simulink model "Controller"  (R2023b)
settings: Solver=FixedStepDiscrete  StartTime=0.0  StopTime=10.0  FixedStep=1e-4  RelTol=1e-3
libraries: mcbcontrolslib x12, slpidlib x3, mcbpositiondecoderlib x2
settings Model: DataDictionary=Controller.sldd  Creator=84339  LastModifiedBy=84339
settings OptimizationCC: DefaultParameterBehavior=Inlined  EnhancedBackFolding=on  PassReuseOutputArgsAs=Individual arguments  ZeroExternalMemoryAtStartup=off  ZeroInternalMemoryAtStartup=off  OptimizeBlockOrder=speed  DifferentSizesBufferReuse=on  OptimizationCustomize=off  EfficientTunableParamExpr=on
settings DebuggingCC: ParameterTunabilityLossMsg=error
settings SFSimCC: MATLABDynamicMemAlloc=off
settings RTWCC: Description=Embedded Coder  SystemTargetFile=ert.tlc  EmbeddedCoderDictionary=Arch.sldd  GenCodeOnly=on  TemplateMakefile=ert_default_tmf
settings CodeAppCC: ForceParamTrailComments=on  IgnoreCustomStorageClasses=off  OperatorAnnotations=on  SimulinkDataObjDesc=on  SFDataObjDesc=on  InsertBlockDesc=on
settings ERTTargetCC: TargetLangStandard=C99 (ISO)  GenerateSampleERTMain=on  InlinedParameterPlacement=NonHierarchical  ERTCustomFileTemplate=example_file_process.tlc

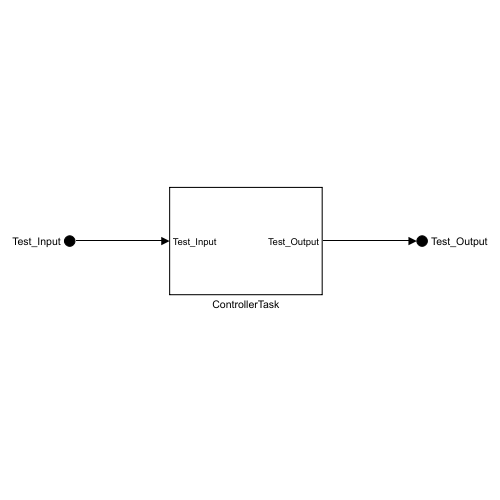
[thumbnail: Simulink's stored preview of the top-level diagram]
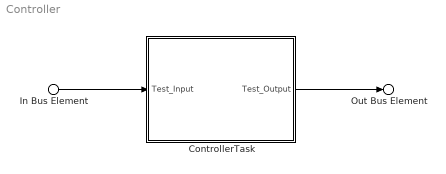
== system Controller ==
  In Bus Element : Inport  PortName=Test_Input
  ControllerTask : Subsystem
  Out Bus Element : Outport  PortName=Test_Output
  wires:
  ControllerTask/1(Test_Output) -> Out Bus Element/1
  In Bus Element/1 -> ControllerTask/1(Test_Input)

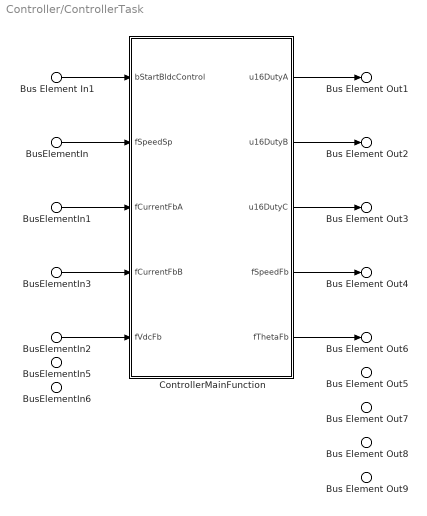
== system Controller/ControllerTask ==
  Bus Element In1 : Inport  PortName=Test_Input  Element=Input1
  BusElementIn : Inport  PortName=Test_Input  Element=Input2
  BusElementIn1 : Inport  PortName=Test_Input  Element=Input3
  BusElementIn3 : Inport  PortName=Test_Input  Element=Input4
  BusElementIn2 : Inport  PortName=Test_Input  Element=Input5
  BusElementIn5 : Inport  PortName=Test_Input  Element=Input6
  BusElementIn6 : Inport  PortName=Test_Input  Element=Input7
  ControllerMainFunction : Subsystem
  Bus Element Out1 : Outport  PortName=Test_Output  Element=Output1
  Bus Element Out2 : Outport  PortName=Test_Output  Element=Output2
  Bus Element Out3 : Outport  PortName=Test_Output  Element=Output3
  Bus Element Out4 : Outport  PortName=Test_Output  Element=Output4
  Bus Element Out5 : Outport  PortName=Test_Output  Element=Output6
  Bus Element Out7 : Outport  PortName=Test_Output  Element=Output7
  Bus Element Out8 : Outport  PortName=Test_Output  Element=Output8
  Bus Element Out9 : Outport  PortName=Test_Output  Element=Output9
  Bus Element Out6 : Outport  PortName=Test_Output  Element=Output5
  wires:
  ControllerMainFunction/1(u16DutyA) -> Bus Element Out1/1
  Bus Element In1/1 -> ControllerMainFunction/1(bStartBldcControl)
  BusElementIn/1 -> ControllerMainFunction/2(fSpeedSp)
  BusElementIn1/1 -> ControllerMainFunction/3(fCurrentFbA)
  BusElementIn3/1 -> ControllerMainFunction/4(fCurrentFbB)
  BusElementIn2/1 -> ControllerMainFunction/5(fVdcFb)
  ControllerMainFunction/2(u16DutyB) -> Bus Element Out2/1
  ControllerMainFunction/3(u16DutyC) -> Bus Element Out3/1
  ControllerMainFunction/4(fSpeedFb) -> Bus Element Out4/1
  ControllerMainFunction/5(fThetaFb) -> Bus Element Out6/1

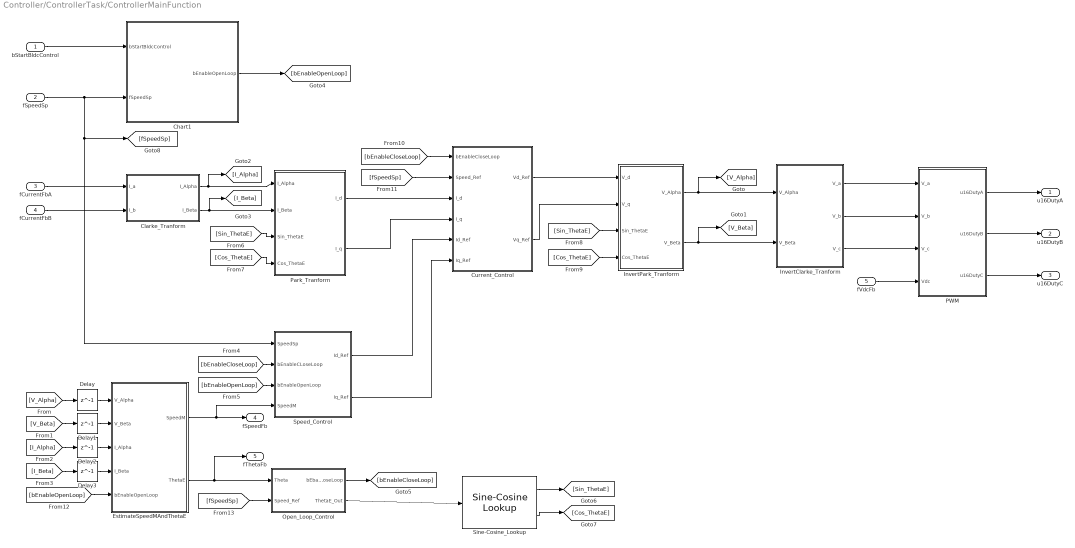
== system Controller/ControllerTask/ControllerMainFunction ==
  bStartBldcControl : Inport
  fSpeedSp : Inport  Port=2
  fCurrentFbA : Inport  Port=3
  fCurrentFbB : Inport  Port=4
  fVdcFb : Inport  Port=5
  Chart1 : Stateflow chart  TreatAsAtomicUnit=on
  Clarke_Tranform : Subsystem
  Current_Control : Subsystem
  Delay{,1..3} (4 alike) : Delay  DelayLength=1
  EstimateSpeedMAndThetaE : Subsystem
  InvertClarke_Tranform : Subsystem
  InvertPark_Tranform : Subsystem
  Open_Loop_Control : Subsystem
  PWM : Subsystem
      settings: RTWFcnNameOpts=Use subsystem name  RTWFileNameOpts=Use subsystem name
  Park_Tranform : Subsystem
  Sine-Cosine_Lookup : mcbcontrolslib/Sine-Cosine Lookup  AngleInput=Per-unit  N_points=1024
  Speed_Control : Subsystem
  u16DutyA : Outport
  u16DutyB : Outport  Port=2
  u16DutyC : Outport  Port=3
  fSpeedFb : Outport  Port=4
  fThetaFb : Outport  Port=5
  wires:
  InvertPark_Tranform/1(V_Alpha) -> [V_Alpha], InvertClarke_Tranform/1(V_Alpha)
  Delay1/1 -> EstimateSpeedMAndThetaE/2(V_Beta)
  [bEnableOpenLoop] -> Speed_Control/3(bEnableOpenLoop)
  PWM/3(u16DutyC) -> u16DutyC/1
  InvertClarke_Tranform/3(V_c) -> PWM/3(V_c)
  Delay/1 -> EstimateSpeedMAndThetaE/1(V_Alpha)
  [V_Alpha] -> Delay/1
  Speed_Control/1(Id_Ref) -> Current_Control/5(Id_Ref)
  fCurrentFbA/1 -> Clarke_Tranform/1(I_a)
  EstimateSpeedMAndThetaE/2(ThetaE) -> fThetaFb/1, Open_Loop_Control/1(Theta)
  [Cos_ThetaE] -> Park_Tranform/4(Cos_ThetaE)
  Delay2/1 -> EstimateSpeedMAndThetaE/3(I_Alpha)
  Sine-Cosine_Lookup/1 -> [Sin_ThetaE]
  Clarke_Tranform/2(I_Beta) -> Park_Tranform/2(I_Beta), [I_Beta]
  [fSpeedSp] -> Current_Control/2(Speed_Ref)
  [bEnableCloseLoop] -> Current_Control/1(bEnableCloseLoop)
  Clarke_Tranform/1(I_Alpha) -> Park_Tranform/1(I_Alpha), [I_Alpha]
  Park_Tranform/1(I_d) -> Current_Control/3(I_d)
  InvertPark_Tranform/2(V_Beta) -> [V_Beta], InvertClarke_Tranform/2(V_Beta)
  InvertClarke_Tranform/1(V_a) -> PWM/1(V_a)
  Chart1/1(bEnableOpenLoop) -> [bEnableOpenLoop]
  fCurrentFbB/1 -> Clarke_Tranform/2(I_b)
  InvertClarke_Tranform/2(V_b) -> PWM/2(V_b)
  Delay3/1 -> EstimateSpeedMAndThetaE/4(I_Beta)
  [Sin_ThetaE] -> InvertPark_Tranform/3(Sin_ThetaE)
  Park_Tranform/2(I_q) -> Current_Control/4(I_q)
  PWM/2(u16DutyB) -> u16DutyB/1
  PWM/1(u16DutyA) -> u16DutyA/1
  Open_Loop_Control/1(bEbableCloseLoop) -> [bEnableCloseLoop]
  fVdcFb/1 -> PWM/4(Vdc)
  [bEnableOpenLoop] -> EstimateSpeedMAndThetaE/5(bEnableOpenLoop)
  [V_Beta] -> Delay1/1
  [bEnableCloseLoop] -> Speed_Control/2(bEnableCLoseLoop)
  [Sin_ThetaE] -> Park_Tranform/3(Sin_ThetaE)
  [Cos_ThetaE] -> InvertPark_Tranform/4(Cos_ThetaE)
  fSpeedSp/1 -> [fSpeedSp], Speed_Control/1(SpeedSp), Chart1/2(fSpeedSp)
  EstimateSpeedMAndThetaE/1(SpeedM) -> Speed_Control/4(SpeedM), fSpeedFb/1
  Open_Loop_Control/2(ThetaE_Out) -> Sine-Cosine_Lookup/1
  Current_Control/2(Vq_Ref) -> InvertPark_Tranform/2(V_q)
  [fSpeedSp] -> Open_Loop_Control/2(Speed_Ref)
  [I_Alpha] -> Delay2/1
  [I_Beta] -> Delay3/1
  Current_Control/1(Vd_Ref) -> InvertPark_Tranform/1(V_d)
  Sine-Cosine_Lookup/2 -> [Cos_ThetaE]
  Speed_Control/2(Iq_Ref) -> Current_Control/6(Iq_Ref)
  bStartBldcControl/1 -> Chart1/1(bStartBldcControl)

== system Controller/ControllerTask/ControllerMainFunction/Clarke_Tranform ==
  I_a : Inport
  I_b : Inport  Port=2
  Clarke Transform : mcbcontrolslib/Clarke Transform  VariantControl=Variant2  PhaseInput=Two inputs  EnPowerInv=off
  I_Alpha : Outport
  I_Beta : Outport  Port=2
  wires:
  Clarke Transform/2 -> I_Beta/1
  I_a/1 -> Clarke Transform/1
  Clarke Transform/1 -> I_Alpha/1
  I_b/1 -> Clarke Transform/2

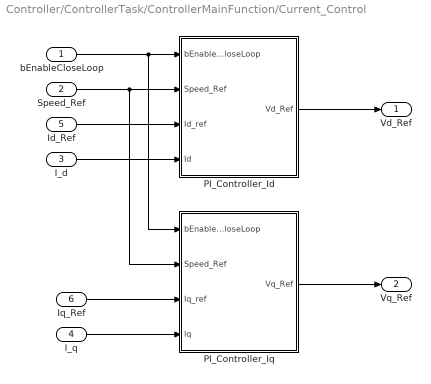
== system Controller/ControllerTask/ControllerMainFunction/Current_Control ==
  bEnableCloseLoop : Inport
  Speed_Ref : Inport  Port=2
  I_d : Inport  Port=3
  I_q : Inport  Port=4
  Id_Ref : Inport  Port=5
  Iq_Ref : Inport  Port=6
  PI_Controller_Id : Subsystem
  PI_Controller_Iq : Subsystem
  Vd_Ref : Outport
  Vq_Ref : Outport  Port=2
  wires:
  PI_Controller_Id/1(Vd_Ref) -> Vd_Ref/1
  bEnableCloseLoop/1 -> PI_Controller_Iq/1(bEnableCloseLoop), PI_Controller_Id/1(bEnableCloseLoop)
  Speed_Ref/1 -> PI_Controller_Iq/2(Speed_Ref), PI_Controller_Id/2(Speed_Ref)
  I_d/1 -> PI_Controller_Id/4(Id)
  Id_Ref/1 -> PI_Controller_Id/3(Id_ref)
  PI_Controller_Iq/1(Vq_Ref) -> Vq_Ref/1
  Iq_Ref/1 -> PI_Controller_Iq/3(Iq_ref)
  I_q/1 -> PI_Controller_Iq/4(Iq)

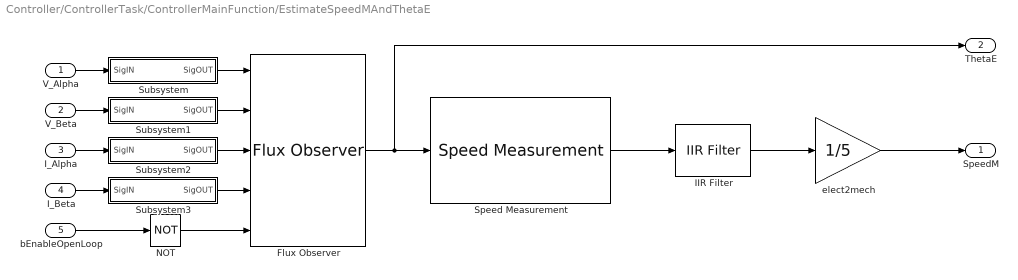
== system Controller/ControllerTask/ControllerMainFunction/EstimateSpeedMAndThetaE ==
  V_Alpha : Inport
  V_Beta : Inport  Port=2
  I_Alpha : Inport  Port=3
  I_Beta : Inport  Port=4
  bEnableOpenLoop : Inport  Port=5
  Flux Observer : mcbpositiondecoderlib/Flux Observer  MotorSelection=PMSM  DataTypeSelect=off  BlockInputUnit=Per-unit  PerUnitVoltage=24/sqrt(3)  PerUnitCurrent=7.77  PositionSelect=on  FluxSelect=off  TorqueSelect=off  PolePairs=4  StatorResistance=2.59  StatorDAxisInductance=0.5e-3  StatorLeakageInductance=0.0068  RotorLeakageInductance=0.0068  MagnetizingInductance=0.0300  CutoffFreq=3.1863  BlockSampleTime=1e-4  PositionUnit=Per-unit  PositionDatatype=single  FluxUnit=Weber  PerUnitFlux=0.1  FluxDatatype=single  TorqueUnit=Nm  PerUnitTorque=100  TorqueDatatype=single  DataType=0
  IIR Filter : mcbcontrolslib/IIR Filter  VariantControl=Low Pass Filter  VariantSelect=Low-pass  Filter_constant=0.01  advancedSettings=off  Ts=50e-6  cutOff_freq=32.1525
  NOT : Logic  Operator=NOT  IconShape=distinctive  AllPortsSameDT=off  OutDataTypeStr=boolean
  Speed Measurement : mcbpositiondecoderlib/Speed Measurement  PositionUnit=Per unit  PositionScalingDatatype=uint32  SpeedCalculationMode=Time interval for speed calculation  SampleTimeAsync=1e-4  MaximumApplicationSpeed=60000  SpeedResolution=5e-6  DelayLength=10  MaximumMeasurableSpeed=29999  MeasurableSpeedResolution=1.397e-05  SpeedUnit=Per unit based on dialog  PerUnitSpeed=2000  SpeedDataType=single
  Subsystem : Subsystem
  Subsystem1 : Subsystem
  Subsystem2 : Subsystem
  Subsystem3 : Subsystem
  elect2mech : Gain  Gain=1/5  RndMeth=Simplest  OutDataTypeStr=Inherit: Same as input
  SpeedM : Outport
  ThetaE : Outport  Port=2
  wires:
  Speed Measurement/1 -> IIR Filter/1
  Flux Observer/1 -> Speed Measurement/1, ThetaE/1
  bEnableOpenLoop/1 -> NOT/1
  NOT/1 -> Flux Observer/5
  I_Beta/1 -> Subsystem3/1(SigIN)
  I_Alpha/1 -> Subsystem2/1(SigIN)
  V_Beta/1 -> Subsystem1/1(SigIN)
  V_Alpha/1 -> Subsystem/1(SigIN)
  Subsystem/1(SigOUT) -> Flux Observer/1
  Subsystem1/1(SigOUT) -> Flux Observer/2
  Subsystem2/1(SigOUT) -> Flux Observer/3
  Subsystem3/1(SigOUT) -> Flux Observer/4
  IIR Filter/1 -> elect2mech/1
  elect2mech/1 -> SpeedM/1

== system Controller/ControllerTask/ControllerMainFunction/InvertClarke_Tranform ==
  V_Alpha : Inport
  V_Beta : Inport  Port=2
  Inverse Clarke Transform : mcbcontrolslib/Inverse Clarke Transform  PhaseInput=Two inputs  EnPowerInv=off
      settings: LibrarySourceBlock=mcblib/Controls/Math Transforms/Inverse Clarke Transform
  V_a : Outport
  V_b : Outport  Port=2
  V_c : Outport  Port=3
  wires:
  V_Alpha/1 -> Inverse Clarke Transform/1
  V_Beta/1 -> Inverse Clarke Transform/2
  Inverse Clarke Transform/2 -> V_b/1
  Inverse Clarke Transform/1 -> V_a/1
  Inverse Clarke Transform/3 -> V_c/1

== system Controller/ControllerTask/ControllerMainFunction/InvertPark_Tranform ==
  V_d : Inport
  V_q : Inport  Port=2
  Sin_ThetaE : Inport  Port=3
  Cos_ThetaE : Inport  Port=4
  Inverse Park Transform : mcbcontrolslib/Inverse Park Transform  PhaseInput=Two inputs  AxisAlignment=D-axis  ThetaInput=Sine and Cosine electrical position  AngleInput=Per-unit  N_points=1024
  V_Alpha : Outport
  V_Beta : Outport  Port=2
  wires:
  V_d/1 -> Inverse Park Transform/1
  V_q/1 -> Inverse Park Transform/2
  Sin_ThetaE/1 -> Inverse Park Transform/3
  Cos_ThetaE/1 -> Inverse Park Transform/4
  Inverse Park Transform/2 -> V_Beta/1
  Inverse Park Transform/1 -> V_Alpha/1

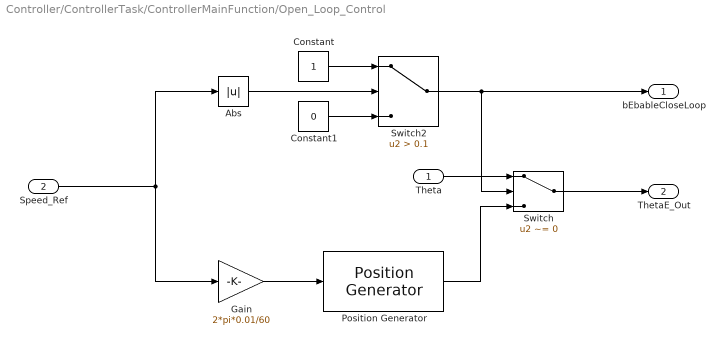
== system Controller/ControllerTask/ControllerMainFunction/Open_Loop_Control ==
  Theta : Inport
  Speed_Ref : Inport  Port=2
  Abs : Abs  SaturateOnIntegerOverflow=off
  Constant : Constant  OutDataTypeStr=boolean
  Constant1 : Constant  Value=0  OutDataTypeStr=boolean
  Gain : Gain  Gain=2*pi*0.01/60  OutDataTypeStr=Inherit: Same as input  ParamDataTypeStr=Inherit: Same as input
  Position Generator : mcbcontrolslib/Position Generator  AngleOutput=Per-unit  ExternalReset=none  Offset=0
  Switch : Switch  Criteria=u2 ~= 0  Threshold=0.1  SaturateOnIntegerOverflow=off  InputSameDT=off
  Switch2 : Switch  Criteria=u2 > Threshold  Threshold=0.1  SaturateOnIntegerOverflow=off  InputSameDT=off
  bEbableCloseLoop : Outport
  ThetaE_Out : Outport  Port=2
  wires:
  Constant1/1 -> Switch2/3
  Constant/1 -> Switch2/1
  Abs/1 -> Switch2/2
  Theta/1 -> Switch/1
  Switch/1 -> ThetaE_Out/1
  Gain/1 -> Position Generator/1
  Speed_Ref/1 -> Abs/1, Gain/1
  Switch2/1 -> Switch/2, bEbableCloseLoop/1
  Position Generator/1 -> Switch/3

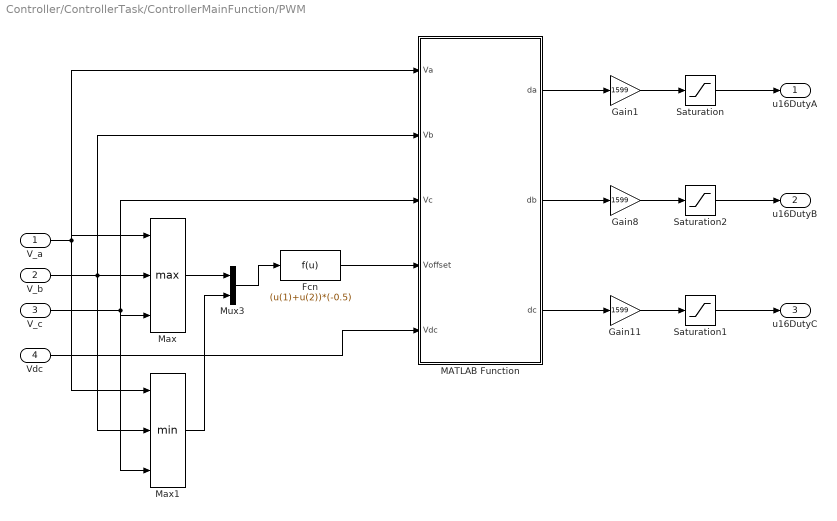
== system Controller/ControllerTask/ControllerMainFunction/PWM ==
  V_a : Inport
  V_b : Inport  Port=2
  V_c : Inport  Port=3
  Vdc : Inport  Port=4
  Fcn : Fcn  Expr=(u(1)+u(2))*(-0.5)
  Gain1 : Gain  Gain=1599  OutDataTypeStr=uint16
  Gain11 : Gain  Gain=1599  OutDataTypeStr=uint16
  Gain8 : Gain  Gain=1599  OutDataTypeStr=uint16
  MATLAB Function : MATLAB Function  TreatAsAtomicUnit=on
  Max : MinMax  Function=max  Inputs=3
  Max1 : MinMax  Inputs=3
  Mux3 : Mux  Inputs=2
  Saturation : Saturate  UpperLimit=1599  LowerLimit=0
  Saturation1 : Saturate  UpperLimit=1599  LowerLimit=0
  Saturation2 : Saturate  UpperLimit=1599  LowerLimit=0
  u16DutyA : Outport
  u16DutyB : Outport  Port=2
  u16DutyC : Outport  Port=3
  wires:
  Saturation1/1 -> u16DutyC/1
  Fcn/1 -> MATLAB Function/4(Voffset)
  Mux3/1 -> Fcn/1
  MATLAB Function/2(db) -> Gain8/1
  Max1/1 -> Mux3/2
  Saturation2/1 -> u16DutyB/1
  Gain8/1 -> Saturation2/1
  MATLAB Function/1(da) -> Gain1/1
  MATLAB Function/3(dc) -> Gain11/1
  Saturation/1 -> u16DutyA/1
  Gain11/1 -> Saturation1/1
  Max/1 -> Mux3/1
  Gain1/1 -> Saturation/1
  V_a/1 -> MATLAB Function/1(Va), Max1/1, Max/1
  V_b/1 -> MATLAB Function/2(Vb), Max1/2, Max/2
  V_c/1 -> MATLAB Function/3(Vc), Max1/3, Max/3
  Vdc/1 -> MATLAB Function/5(Vdc)

== system Controller/ControllerTask/ControllerMainFunction/Park_Tranform ==
  I_Alpha : Inport
  I_Beta : Inport  Port=2
  Sin_ThetaE : Inport  Port=3
  Cos_ThetaE : Inport  Port=4
  Park Transform : mcbcontrolslib/Park Transform  PhaseInput=Two inputs  AxisAlignment=D-axis  ThetaInput=Sine and Cosine electrical position  AngleInput=Per-unit  N_points=1024
      settings: LibrarySourceBlock=mcbhdllib/Controls/Math Transforms/Park Transform
  I_d : Outport
  I_q : Outport  Port=2
  wires:
  Park Transform/2 -> I_q/1
  I_Alpha/1 -> Park Transform/1
  Park Transform/1 -> I_d/1
  I_Beta/1 -> Park Transform/2
  Sin_ThetaE/1 -> Park Transform/3
  Cos_ThetaE/1 -> Park Transform/4

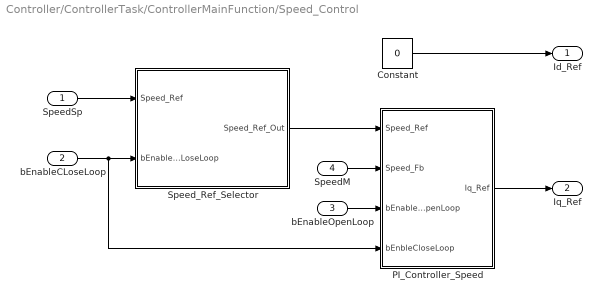
== system Controller/ControllerTask/ControllerMainFunction/Speed_Control ==
  SpeedSp : Inport
  bEnableCLoseLoop : Inport  Port=2
  bEnableOpenLoop : Inport  Port=3
  SpeedM : Inport  Port=4
  Constant : Constant  Value=0  OutDataTypeStr=single
  PI_Controller_Speed : Subsystem
  Speed_Ref_Selector : Subsystem
  Id_Ref : Outport
  Iq_Ref : Outport  Port=2
  wires:
  Constant/1 -> Id_Ref/1
  PI_Controller_Speed/1(Iq_Ref) -> Iq_Ref/1
  SpeedSp/1 -> Speed_Ref_Selector/1(Speed_Ref)
  bEnableCLoseLoop/1 -> PI_Controller_Speed/4(bEnbleCloseLoop), Speed_Ref_Selector/2(bEnableCLoseLoop)
  Speed_Ref_Selector/1(Speed_Ref_Out) -> PI_Controller_Speed/1(Speed_Ref)
  SpeedM/1 -> PI_Controller_Speed/2(Speed_Fb)
  bEnableOpenLoop/1 -> PI_Controller_Speed/3(bEnableOpenLoop)

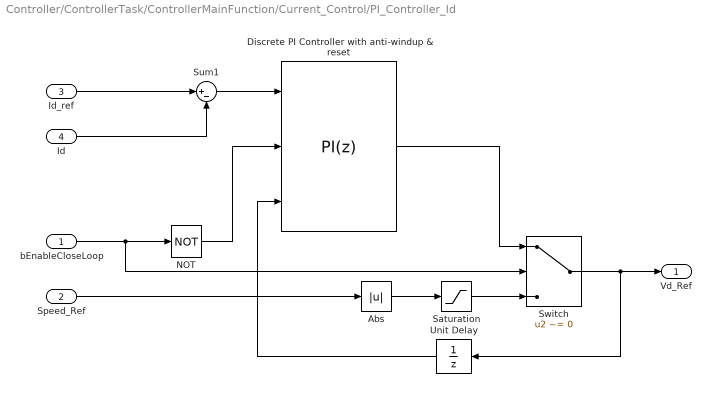
== system Controller/ControllerTask/ControllerMainFunction/Current_Control/PI_Controller_Id ==
  bEnableCloseLoop : Inport
  Speed_Ref : Inport  Port=2
  Id_ref : Inport  Port=3
  Id : Inport  Port=4
  Abs : Abs  RndMeth=Simplest  SaturateOnIntegerOverflow=off
  Discrete PI Controller with anti-windup & reset : slpidlib/PID Controller  Controller=PI  Form=Parallel  TimeDomain=Discrete-time  UseExternalTs=off  SampleTime=-1  IntegratorMethod=Forward Euler  FilterMethod=Forward Euler  ControllerParametersSource=internal  P=0.1  I=0.01  UseKiTs=on  D=0  N=100  UseFilter=on  TunerSelectOption=Transfer Function Based (PID Tuner App)  InitialConditionSource=external  InitialConditionForIntegrator=0  InitialConditionForFilter=0  DifferentiatorICPrevScaledInput=0  ExternalReset=level  TrackingMode=off  Kt=1  LimitOutput=on  SatLimitsSource=internal  UpperSaturationLimit=24/sqrt(3)  LowerSaturationLimit=-24/sqrt(3)  LinearizeAsGain=on  AntiWindupMode=clamping  Kb=1  LimitIntegrator=off  UpperIntegratorSaturationLimit=inf  LowerIntegratorSaturationLimit=-inf  RndMeth=Simplest  POutMin=[]  POutMax=[]  IOutMin=[]  IOutMax=[]  DOutMin=[]  DOutMax=[]  NOutMin=[]  NOutMax=[]  SumOutMin=[]  SumOutMax=[]  SaturationOutDataTypeStr=Inherit: Inherit via back propagation  SaturationOutMin=[]  SaturationOutMax=[]  PParamMin=[]  PParamMax=[]  IParamMin=[]  IParamMax=[]  DParamMin=[]  DParamMax=[]  NParamMin=[]  NParamMax=[]  KbParamMin=[]  KbParamMax=[]  KtParamMin=[]  KtParamMax=[]  KbOutMin=[]  KbOutMax=[]  KtOutMin=[]  KtOutMax=[]  IntegratorOutMin=[]  IntegratorOutMax=[]  FilterOutMin=[]  FilterOutMax=[]  SumI1OutMin=[]  SumI1OutMax=[]  SumI2OutMin=[]  SumI2OutMax=[]  SumI3OutMin=[]  SumI3OutMax=[]  SumI4OutMin=[]  SumI4OutMax=[]  SumDOutMin=[]  SumDOutMax=[]  DifferentiatorOutMin=[]  DifferentiatorOutMax=[]  FilterDiffOutCoefMin=[]  FilterDiffOutCoefMax=[]  ReciprocalOutMin=[]  ReciprocalOutMax=[]  SumDenOutMin=[]  SumDenOutMax=[]  SumNumOutMin=[]  SumNumOutMax=[]  DivideOutMin=[]  DivideOutMax=[]  UdiffTsProdOutMin=[]  UdiffTsProdOutMax=[]  NTsProdOutMin=[]  NTsProdOutMax=[]  UintegralTsProdOutMin=[]  UintegralTsProdOutMax=[]  UngainTsProdOutMin=[]  UngainTsProdOutMax=[]  ClampingZeroOutDataTypeStr=Inherit: Inherit via back propagation  ClampingZeroOutMin=[]  ClampingZeroOutMax=[]  FilterDenConstantOutDataTypeStr=Inherit: Inherit via back propagation  FilterDenConstantOutMin=[]  FilterDenConstantOutMax=[]  PCopyOutDataTypeStr=Inherit: Inherit via back propagation  PCopyOutMin=[]  PCopyOutMax=[]  NCopyOutDataTypeStr=Inherit: Inherit via back propagation  NCopyOutMin=[]  NCopyOutMax=[]  IntegratorContinuousStateAttributes=''  IntegratorStateMustResolveToSignalObject=off  IntegratorRTWStateStorageClass=Auto  FilterContinuousStateAttributes=''  FilterStateMustResolveToSignalObject=off  FilterRTWStateStorageClass=Auto  ParallelPVariant=InternalParameters  IdealPVariant=Disabled  IVariant=InternalParameters  DVariant=Disabled  IntegratorVariant=Discrete  SatVariant=Enabled  AWVariant=DiscClampingParallel  PCopyVariant=Disabled  TRVariant=Disabled  FdbkBlocksVariant=Forward  IdealPFdbkVariant=Disabled  SatFdbkVariant=Disabled  DerivativeFilterVariant=Disabled  NVariant=Disabled  NCopyVariant=Disabled_SignalSpec  FilterICVariant=Disabled  IntegratorICVariant=ExternalICs  ExternalResetVariant=ExternalReset  TRSumVariant=Passthrough  SumFdbkVariant=Disabled  SumVariant=Sum_PI  TsampFilterVariant=InternalTs  TsampNgainVariant=Passthrough  TsampIntegralVariant=Disabled_SignalSpec  ExternalSaturationOutDataTypeStr=Inherit: Same as second input
      settings: LibrarySourceBlock=mcbcontrolslib/PI Controller
  NOT : Logic  Operator=NOT  IconShape=distinctive  AllPortsSameDT=off  OutDataTypeStr=boolean
  Saturation : Saturate  UpperLimit=95.5*2  LowerLimit=95.5  RndMeth=Simplest
  Sum1 : Sum  Inputs=|+-
  Switch : Switch  Criteria=u2 ~= 0  RndMeth=Simplest  SaturateOnIntegerOverflow=off  InputSameDT=off
  Unit Delay : UnitDelay  SampleTime=-1  HasFrameUpgradeWarning=on
  Vd_Ref : Outport  VectorParamsAs1DForOutWhenUnconnected=off
  wires:
  Switch/1 -> Unit Delay/1, Vd_Ref/1
  Id/1 -> Sum1/2
  Sum1/1 -> Discrete PI Controller with anti-windup & reset/1
  Id_ref/1 -> Sum1/1
  NOT/1 -> Discrete PI Controller with anti-windup & reset/2
  Unit Delay/1 -> Discrete PI Controller with anti-windup & reset/3
  Discrete PI Controller with anti-windup & reset/1 -> Switch/1
  bEnableCloseLoop/1 -> Switch/2, NOT/1
  Saturation/1 -> Switch/3
  Abs/1 -> Saturation/1
  Speed_Ref/1 -> Abs/1

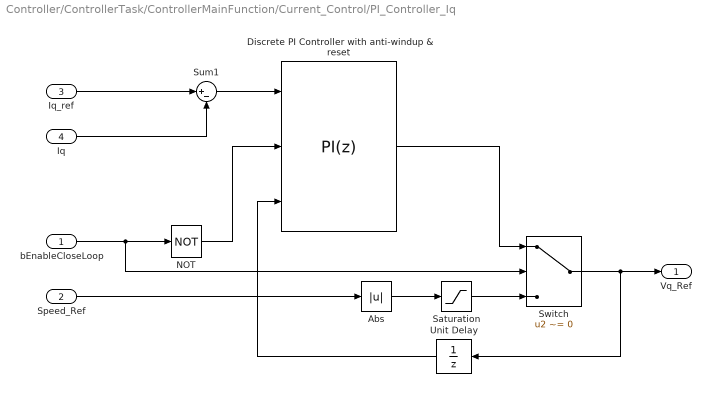
== system Controller/ControllerTask/ControllerMainFunction/Current_Control/PI_Controller_Iq ==
  bEnableCloseLoop : Inport
  Speed_Ref : Inport  Port=2
  Iq_ref : Inport  Port=3
  Iq : Inport  Port=4
  Abs : Abs  RndMeth=Simplest  SaturateOnIntegerOverflow=off
  Discrete PI Controller with anti-windup & reset : slpidlib/PID Controller  Controller=PI  Form=Parallel  TimeDomain=Discrete-time  UseExternalTs=off  SampleTime=-1  IntegratorMethod=Forward Euler  FilterMethod=Forward Euler  ControllerParametersSource=internal  P=0.1  I=0.01  UseKiTs=on  D=0  N=100  UseFilter=on  TunerSelectOption=Transfer Function Based (PID Tuner App)  InitialConditionSource=external  InitialConditionForIntegrator=0  InitialConditionForFilter=0  DifferentiatorICPrevScaledInput=0  ExternalReset=level  TrackingMode=off  Kt=1  LimitOutput=on  SatLimitsSource=internal  UpperSaturationLimit=24/sqrt(3)  LowerSaturationLimit=-24/sqrt(3)  LinearizeAsGain=on  AntiWindupMode=clamping  Kb=1  LimitIntegrator=off  UpperIntegratorSaturationLimit=inf  LowerIntegratorSaturationLimit=-inf  RndMeth=Simplest  POutMin=[]  POutMax=[]  IOutMin=[]  IOutMax=[]  DOutMin=[]  DOutMax=[]  NOutMin=[]  NOutMax=[]  SumOutMin=[]  SumOutMax=[]  SaturationOutDataTypeStr=Inherit: Inherit via back propagation  SaturationOutMin=[]  SaturationOutMax=[]  PParamMin=[]  PParamMax=[]  IParamMin=[]  IParamMax=[]  DParamMin=[]  DParamMax=[]  NParamMin=[]  NParamMax=[]  KbParamMin=[]  KbParamMax=[]  KtParamMin=[]  KtParamMax=[]  KbOutMin=[]  KbOutMax=[]  KtOutMin=[]  KtOutMax=[]  IntegratorOutMin=[]  IntegratorOutMax=[]  FilterOutMin=[]  FilterOutMax=[]  SumI1OutMin=[]  SumI1OutMax=[]  SumI2OutMin=[]  SumI2OutMax=[]  SumI3OutMin=[]  SumI3OutMax=[]  SumI4OutMin=[]  SumI4OutMax=[]  SumDOutMin=[]  SumDOutMax=[]  DifferentiatorOutMin=[]  DifferentiatorOutMax=[]  FilterDiffOutCoefMin=[]  FilterDiffOutCoefMax=[]  ReciprocalOutMin=[]  ReciprocalOutMax=[]  SumDenOutMin=[]  SumDenOutMax=[]  SumNumOutMin=[]  SumNumOutMax=[]  DivideOutMin=[]  DivideOutMax=[]  UdiffTsProdOutMin=[]  UdiffTsProdOutMax=[]  NTsProdOutMin=[]  NTsProdOutMax=[]  UintegralTsProdOutMin=[]  UintegralTsProdOutMax=[]  UngainTsProdOutMin=[]  UngainTsProdOutMax=[]  ClampingZeroOutDataTypeStr=Inherit: Inherit via back propagation  ClampingZeroOutMin=[]  ClampingZeroOutMax=[]  FilterDenConstantOutDataTypeStr=Inherit: Inherit via back propagation  FilterDenConstantOutMin=[]  FilterDenConstantOutMax=[]  PCopyOutDataTypeStr=Inherit: Inherit via back propagation  PCopyOutMin=[]  PCopyOutMax=[]  NCopyOutDataTypeStr=Inherit: Inherit via back propagation  NCopyOutMin=[]  NCopyOutMax=[]  IntegratorContinuousStateAttributes=''  IntegratorStateMustResolveToSignalObject=off  IntegratorRTWStateStorageClass=Auto  FilterContinuousStateAttributes=''  FilterStateMustResolveToSignalObject=off  FilterRTWStateStorageClass=Auto  ParallelPVariant=InternalParameters  IdealPVariant=Disabled  IVariant=InternalParameters  DVariant=Disabled  IntegratorVariant=Discrete  SatVariant=Enabled  AWVariant=DiscClampingParallel  PCopyVariant=Disabled  TRVariant=Disabled  FdbkBlocksVariant=Forward  IdealPFdbkVariant=Disabled  SatFdbkVariant=Disabled  DerivativeFilterVariant=Disabled  NVariant=Disabled  NCopyVariant=Disabled_SignalSpec  FilterICVariant=Disabled  IntegratorICVariant=ExternalICs  ExternalResetVariant=ExternalReset  TRSumVariant=Passthrough  SumFdbkVariant=Disabled  SumVariant=Sum_PI  TsampFilterVariant=InternalTs  TsampNgainVariant=Passthrough  TsampIntegralVariant=Disabled_SignalSpec  ExternalSaturationOutDataTypeStr=Inherit: Same as second input
      settings: LibrarySourceBlock=mcbcontrolslib/PI Controller
  NOT : Logic  Operator=NOT  IconShape=distinctive  AllPortsSameDT=off  OutDataTypeStr=boolean
  Saturation : Saturate  UpperLimit=95.5*2  LowerLimit=95.5  RndMeth=Simplest
  Sum1 : Sum  Inputs=|+-
  Switch : Switch  Criteria=u2 ~= 0  RndMeth=Simplest  SaturateOnIntegerOverflow=off  InputSameDT=off
  Unit Delay : UnitDelay  SampleTime=-1  HasFrameUpgradeWarning=on
  Vq_Ref : Outport  VectorParamsAs1DForOutWhenUnconnected=off
  wires:
  Switch/1 -> Unit Delay/1, Vq_Ref/1
  Iq/1 -> Sum1/2
  Sum1/1 -> Discrete PI Controller with anti-windup & reset/1
  Iq_ref/1 -> Sum1/1
  NOT/1 -> Discrete PI Controller with anti-windup & reset/2
  Unit Delay/1 -> Discrete PI Controller with anti-windup & reset/3
  Discrete PI Controller with anti-windup & reset/1 -> Switch/1
  bEnableCloseLoop/1 -> Switch/2, NOT/1
  Saturation/1 -> Switch/3
  Abs/1 -> Saturation/1
  Speed_Ref/1 -> Abs/1

== system Controller/ControllerTask/ControllerMainFunction/EstimateSpeedMAndThetaE/Subsystem ==
  SigIN : Inport
  IIR Filter : mcbcontrolslib/IIR Filter  VariantControl=Low Pass Filter  VariantSelect=Low-pass  Filter_constant=0.005*(1e-4/50e-6)  advancedSettings=off  Ts=50e-6  cutOff_freq=32.1525
  Sum6 : Sum  Inputs=|+-  RndMeth=Simplest  OutDataTypeStr=Inherit: Same as first input
  SigOUT : Outport
  wires:
  SigIN/1 -> Sum6/1, IIR Filter/1
  Sum6/1 -> SigOUT/1
  IIR Filter/1 -> Sum6/2

== system Controller/ControllerTask/ControllerMainFunction/EstimateSpeedMAndThetaE/Subsystem1 ==
  SigIN : Inport
  IIR Filter : mcbcontrolslib/IIR Filter  VariantControl=Low Pass Filter  VariantSelect=Low-pass  Filter_constant=0.005*(1e-4/50e-6)  advancedSettings=off  Ts=50e-6  cutOff_freq=32.1525
  Sum6 : Sum  Inputs=|+-  RndMeth=Simplest  OutDataTypeStr=Inherit: Same as first input
  SigOUT : Outport
  wires:
  SigIN/1 -> Sum6/1, IIR Filter/1
  Sum6/1 -> SigOUT/1
  IIR Filter/1 -> Sum6/2

== system Controller/ControllerTask/ControllerMainFunction/EstimateSpeedMAndThetaE/Subsystem2 ==
  SigIN : Inport
  IIR Filter : mcbcontrolslib/IIR Filter  VariantControl=Low Pass Filter  VariantSelect=Low-pass  Filter_constant=0.005*(1e-4/50e-6)  advancedSettings=off  Ts=50e-6  cutOff_freq=32.1525
  Sum6 : Sum  Inputs=|+-  RndMeth=Simplest  OutDataTypeStr=Inherit: Same as first input
  SigOUT : Outport
  wires:
  SigIN/1 -> Sum6/1, IIR Filter/1
  Sum6/1 -> SigOUT/1
  IIR Filter/1 -> Sum6/2

== system Controller/ControllerTask/ControllerMainFunction/EstimateSpeedMAndThetaE/Subsystem3 ==
  SigIN : Inport
  IIR Filter : mcbcontrolslib/IIR Filter  VariantControl=Low Pass Filter  VariantSelect=Low-pass  Filter_constant=0.005*(1e-4/50e-6)  advancedSettings=off  Ts=50e-6  cutOff_freq=32.1525
  Sum6 : Sum  Inputs=|+-  RndMeth=Simplest  OutDataTypeStr=Inherit: Same as first input
  SigOUT : Outport
  wires:
  SigIN/1 -> Sum6/1, IIR Filter/1
  Sum6/1 -> SigOUT/1
  IIR Filter/1 -> Sum6/2

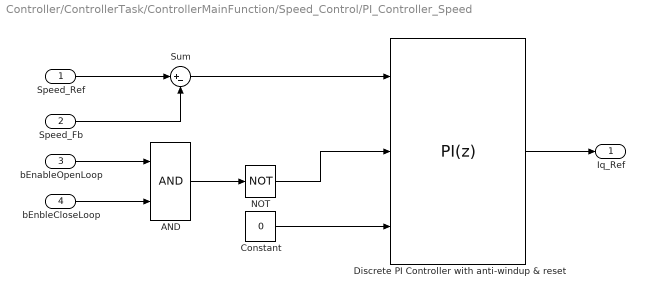
== system Controller/ControllerTask/ControllerMainFunction/Speed_Control/PI_Controller_Speed ==
  Speed_Ref : Inport
  Speed_Fb : Inport  Port=2
  bEnableOpenLoop : Inport  Port=3
  bEnbleCloseLoop : Inport  Port=4
  AND : Logic  AllPortsSameDT=off  OutDataTypeStr=boolean
  Constant : Constant  Value=0  OutDataTypeStr=single
  Discrete PI Controller with anti-windup & reset : slpidlib/PID Controller  Controller=PI  Form=Parallel  TimeDomain=Discrete-time  UseExternalTs=off  SampleTime=-1  IntegratorMethod=Forward Euler  FilterMethod=Forward Euler  ControllerParametersSource=internal  P=0.05  I=0.001  UseKiTs=on  D=0  N=100  UseFilter=on  TunerSelectOption=Transfer Function Based (PID Tuner App)  InitialConditionSource=external  InitialConditionForIntegrator=0  InitialConditionForFilter=0  DifferentiatorICPrevScaledInput=0  ExternalReset=level  TrackingMode=off  Kt=1  LimitOutput=on  SatLimitsSource=internal  UpperSaturationLimit=3/(2*1/5.18)  LowerSaturationLimit=-3/(2*1/5.18)  LinearizeAsGain=on  AntiWindupMode=clamping  Kb=1  LimitIntegrator=off  UpperIntegratorSaturationLimit=inf  LowerIntegratorSaturationLimit=-inf  RndMeth=Simplest  POutMin=[]  POutMax=[]  IOutMin=[]  IOutMax=[]  DOutMin=[]  DOutMax=[]  NOutMin=[]  NOutMax=[]  SumOutMin=[]  SumOutMax=[]  SaturationOutDataTypeStr=Inherit: Inherit via back propagation  SaturationOutMin=[]  SaturationOutMax=[]  PParamMin=[]  PParamMax=[]  IParamMin=[]  IParamMax=[]  DParamMin=[]  DParamMax=[]  NParamMin=[]  NParamMax=[]  KbParamMin=[]  KbParamMax=[]  KtParamMin=[]  KtParamMax=[]  KbOutMin=[]  KbOutMax=[]  KtOutMin=[]  KtOutMax=[]  IntegratorOutMin=[]  IntegratorOutMax=[]  FilterOutMin=[]  FilterOutMax=[]  SumI1OutMin=[]  SumI1OutMax=[]  SumI2OutMin=[]  SumI2OutMax=[]  SumI3OutMin=[]  SumI3OutMax=[]  SumI4OutMin=[]  SumI4OutMax=[]  SumDOutMin=[]  SumDOutMax=[]  DifferentiatorOutMin=[]  DifferentiatorOutMax=[]  FilterDiffOutCoefMin=[]  FilterDiffOutCoefMax=[]  ReciprocalOutMin=[]  ReciprocalOutMax=[]  SumDenOutMin=[]  SumDenOutMax=[]  SumNumOutMin=[]  SumNumOutMax=[]  DivideOutMin=[]  DivideOutMax=[]  UdiffTsProdOutMin=[]  UdiffTsProdOutMax=[]  NTsProdOutMin=[]  NTsProdOutMax=[]  UintegralTsProdOutMin=[]  UintegralTsProdOutMax=[]  UngainTsProdOutMin=[]  UngainTsProdOutMax=[]  ClampingZeroOutDataTypeStr=Inherit: Inherit via back propagation  ClampingZeroOutMin=[]  ClampingZeroOutMax=[]  FilterDenConstantOutDataTypeStr=Inherit: Inherit via back propagation  FilterDenConstantOutMin=[]  FilterDenConstantOutMax=[]  PCopyOutDataTypeStr=Inherit: Inherit via back propagation  PCopyOutMin=[]  PCopyOutMax=[]  NCopyOutDataTypeStr=Inherit: Inherit via back propagation  NCopyOutMin=[]  NCopyOutMax=[]  IntegratorContinuousStateAttributes=''  IntegratorStateMustResolveToSignalObject=off  IntegratorRTWStateStorageClass=Auto  FilterContinuousStateAttributes=''  FilterStateMustResolveToSignalObject=off  FilterRTWStateStorageClass=Auto  ParallelPVariant=InternalParameters  IdealPVariant=Disabled  IVariant=InternalParameters  DVariant=Disabled  IntegratorVariant=Discrete  SatVariant=Enabled  AWVariant=DiscClampingParallel  PCopyVariant=Disabled  TRVariant=Disabled  FdbkBlocksVariant=Forward  IdealPFdbkVariant=Disabled  SatFdbkVariant=Disabled  DerivativeFilterVariant=Disabled  NVariant=Disabled  NCopyVariant=Disabled_SignalSpec  FilterICVariant=Disabled  IntegratorICVariant=ExternalICs  ExternalResetVariant=ExternalReset  TRSumVariant=Passthrough  SumFdbkVariant=Disabled  SumVariant=Sum_PI  TsampFilterVariant=InternalTs  TsampNgainVariant=Passthrough  TsampIntegralVariant=Disabled_SignalSpec  ExternalSaturationOutDataTypeStr=Inherit: Same as second input
      settings: LibrarySourceBlock=mcbcontrolslib/PI Controller
  NOT : Logic  Operator=NOT  IconShape=distinctive  AllPortsSameDT=off  OutDataTypeStr=boolean
  Sum : Sum  Inputs=|+-  OutDataTypeStr=Inherit: Same as first input
  Iq_Ref : Outport  VectorParamsAs1DForOutWhenUnconnected=off
  wires:
  Discrete PI Controller with anti-windup & reset/1 -> Iq_Ref/1
  Speed_Fb/1 -> Sum/2
  Sum/1 -> Discrete PI Controller with anti-windup & reset/1
  NOT/1 -> Discrete PI Controller with anti-windup & reset/2
  Constant/1 -> Discrete PI Controller with anti-windup & reset/3
  bEnableOpenLoop/1 -> AND/1
  bEnbleCloseLoop/1 -> AND/2
  AND/1 -> NOT/1
  Speed_Ref/1 -> Sum/1

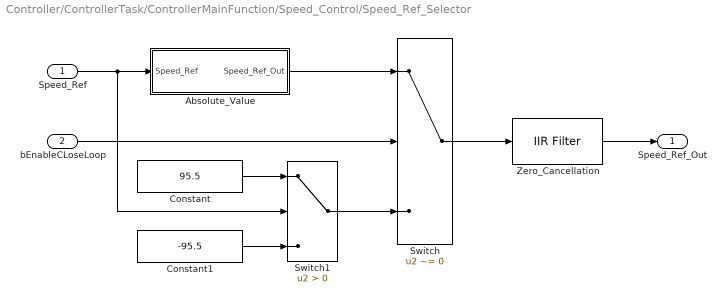
== system Controller/ControllerTask/ControllerMainFunction/Speed_Control/Speed_Ref_Selector ==
  Speed_Ref : Inport
  bEnableCLoseLoop : Inport  Port=2
  Absolute_Value : Subsystem
  Constant : Constant  Value=95.5  OutDataTypeStr=dataType
  Constant1 : Constant  Value=-95.5  OutDataTypeStr=dataType
  Switch : Switch  Criteria=u2 ~= 0  SaturateOnIntegerOverflow=off  InputSameDT=off
  Switch1 : Switch  Criteria=u2 > Threshold  SaturateOnIntegerOverflow=off  InputSameDT=off
  Zero_Cancellation : mcbcontrolslib/IIR Filter  VariantControl=Low Pass Filter  VariantSelect=Low-pass  Filter_constant=0.01  advancedSettings=off  Ts=50e-6  cutOff_freq=32.1525
  Speed_Ref_Out : Outport
  wires:
  bEnableCLoseLoop/1 -> Switch/2
  Constant/1 -> Switch1/1
  Switch1/1 -> Switch/3
  Constant1/1 -> Switch1/3
  Speed_Ref/1 -> Switch1/2, Absolute_Value/1(Speed_Ref)
  Absolute_Value/1(Speed_Ref_Out) -> Switch/1
  Switch/1 -> Zero_Cancellation/1
  Zero_Cancellation/1 -> Speed_Ref_Out/1

== system Controller/ControllerTask/ControllerMainFunction/Speed_Control/Speed_Ref_Selector/Absolute_Value ==
  Speed_Ref : Inport
  Rate Limiter : RateLimiter  RisingSlewLimit=5  FallingSlewLimit=-5  SampleTimeMode=inherited  InitialCondition=95.5
  Rate Limiter1 : RateLimiter  RisingSlewLimit=5  FallingSlewLimit=-5  SampleTimeMode=inherited  InitialCondition=-95.5
  Switch : Switch  SaturateOnIntegerOverflow=off  InputSameDT=off
  Speed_Ref_Out : Outport
  wires:
  Switch/1 -> Speed_Ref_Out/1
  Rate Limiter/1 -> Switch/1
  Rate Limiter1/1 -> Switch/3
  Speed_Ref/1 -> Rate Limiter/1, Switch/2, Rate Limiter1/1

== stateflow chart Controller/ControllerTask/ControllerMainFunction/Chart1 ==
  state Startup
    en:
    bEnableOpenLoop = false;
  state OpenLoop
    en:
    bEnableOpenLoop = true;
  (default) -> Startup
  Startup -> OpenLoop : [bStartBldcControl == true]
  OpenLoop -> Startup : [bStartBldcControl == false]
  data: bStartBldcControl input; fSpeedSp input; bEnableOpenLoop output

== matlab function Controller/ControllerTask/ControllerMainFunction/PWM/MATLAB Function ==
  data: Va input; da output; Vb input; Vc input; Voffset input; db output; dc output; Vdc input
function [da, db, dc] = Calculate_Duty(Va, Vb, Vc, Voffset, Vdc)
da = 0.5 + (Va+Voffset)/Vdc;
db = 0.5 + (Vb+Voffset)/Vdc;
dc = 0.5 + (Vc+Voffset)/Vdc;
